simulink model "QD2_DroneStack_PID_2021a"  (R2022a)
settings: Solver=ode1  StartTime=0.0  StopTime=inf  FixedStep=1/1000  RelTol=1e-3  EnableMultiTasking=on
InitFcn:
  | Motor_Mapping_7_Inch
model workspace (MAT data in the model file):
  target_system = 1
values from neighbouring files (symbols this model uses):
  KT = [0.03616,0.117,-0.01215]    [Motor_Mapping_7_Inch.m]
  Motor_Matrix = [ 0.25   -1/(2*L_Roll)    1/(2*L_Pitch)    K_Tau/4;                  0.25   -1/(2*L_Roll)   -1/(2*L_Pitch)   -K_Tau/4;                  0.25    1/(2*L_Roll)    1/(2*L_Pitch)   -K_Tau/4;                  0.25    1/(2*L_Roll)   -1/(2*L_Pitch)    K_Tau/4]    [Motor_Mapping_7_Inch.m]
undefined symbols (not defined in the file or in its folder): _Commander, _QDrone2, _Stabilizer, datetime, HIL, lf, log_, m, n, qc_get_step_size, s, saved_data
libraries: quarc_library x94, simulink x27, simulink_extras x9
(part 4 of 4)

== matlab function QD2_DroneStack_PID_2021a/COMMANDER (ANGLE MODE)/STATE MACHINE LOGIC ==
  data: E_Abort output; isArm output; pt_ARM_to_TAKEOFF_THROTTLE output; pt_TAKE_OFF_HEIGHT_TO_AUTOLAND output; pt_FLIGHT_TO_AUTOLAND output; current_state input; initializing input; Tracking_Issue input; Communication_Issue input; low_battery input; trigger_1 input; trigger_2 input; E_abort input; joystick_issue input; net_throttle_at_trim input; net_throttle_close_to_zero input; ctrl_throttle_close_to_zero input; take_off_successful input; flying_too_low input; flying_too_high input; close_to_ground input; pt_TAKEOFF_THROTTLE_TO_TAKEOFF_HEIGHT output; pt_TAKE_OFF_HEIGHT_TO_FLIGHT output; pt_AUTOLAND_TO_DISABLE output; pt_EMERGENCY_STOP_TO_DISABLE output; pt_EMERGENCY_ABORT_TO_DISABLE output; Error output; stop_model output; sensor_failed input
function [E_Abort, isArm, pt_ARM_to_TAKEOFF_THROTTLE, pt_TAKE_OFF_HEIGHT_TO_AUTOLAND, pt_FLIGHT_TO_AUTOLAND, pt_TAKEOFF_THROTTLE_TO_TAKEOFF_HEIGHT, pt_TAKE_OFF_HEIGHT_TO_FLIGHT, pt_AUTOLAND_TO_DISABLE, pt_EMERGENCY_STOP_TO_DISABLE, pt_EMERGENCY_ABORT_TO_DISABLE, Error, stop_model]...
    = SM_logic(current_state, initializing, Tracking_Issue, Communication_Issue, low_battery, trigger_1, trigger_2, E_abort, joystick_issue,...
    net_throttle_at_trim, net_throttle_close_to_zero, ctrl_throttle_close_to_zero, take_off_successful, flying_too_low, flying_too_high, close_to_ground, sensor_failed)

% Programmatic Logic Block
%
% Logic for the FSM is generated here based on a variety of signals.
% Mostly, logic to programmatically trigger the transition to either a 
% natural next state, or an Error state, is generated here.
%
% Last modified: March, 2020
%
% INPUTS:
% -------
% current_state = previous state of the FSM-------------------------------------------------- (#)         [1]
% initializing = signal representing that the system is initializing (first 5s + buffer)- - - (bool)      [1]
% comm = communication signal representing MAVLINK connection-------------------------------- (bool)      [1]
% peripheral = signal representing joystick and optitrack connection- - - - - - - - - - - - - (bool)      [2]
% low_battery = signal representing low battery---------------------------------------------- (bool)      [1]
% trigger_1 = trigger representing ARM/DISARM - - - - - - - - - - - - - - - - - - - - - - - - (bool)      [1]
% trigger_2 = trigger representing TAKEOFF/AUTOLAND------------------------------------------ (bool)      [1]
% motors_not_spinning = signal representing the motors not spinning - - - - - - - - - - - - - (bool)      [1]
% net_throttle_at_trim = trim throttle for the application drone ---------------------------- (bool)      [1]
% net_throttle_close_to_zero = net throttle is close to zero in emergency stop mode - - - - - (bool)      [1]
% ctrl_throttle_close_to_zero = ctrl throttle is close to zero in emergency stop mode - - - - (bool)      [1]
% take_off_successful = signal representing whether drone has taken-off successfully -------- (bool)      [1]
% flying_too_low = signal representing whether the drone's height is below threshold and cmd- (bool)      [1]
% flying_too_high = signal representing whether the drone's height is above threshold-------- (bool)      [1]
% close_to_ground = signal representing whether the drone is close to the ground to autoland- (bool)      [1]
% 
% OUTPUTS:
% --------
% Error = Whether an Error is issued or not                                                             (bool)    [1]
% E_Abort = fed through for ease of understanding flow (see STATE MACHINE TRANSITION BLOCK)             (bool)    [1]
% isArm = programmatic transition state                                                                 (bool)    [1]
% takeoff = fed through for ease of understanding flow (see STATE MACHINE TRANSITION BLOCK)             (bool)    [1]
% pt_ARM_to_TAKEOFF_THROTTLE = programmatic transition state BEGIN_STATE_TO_FINAL_STATE                 (bool)    [1]
% pt_TAKEOFF_THROTTLE_TO_TAKEOFF_HEIGHT = programmatic transition state BEGIN_STATE_TO_FINAL_STATE      (bool)    [1]
% pt_TAKE_OFF_HEIGHT_TO_AUTOLAND = programmatic transition state BEGIN_STATE_TO_FINAL_STATE             (bool)    [1]
% pt_TAKEOFF_THROTTLE_TO_TAKEOFF_HEIGHT = programmatic transition state BEGIN_STATE_TO_FINAL_STATE      (bool)    [1]
% pt_TAKE_OFF_HEIGHT_TO_FLIGHT = programmatic transition state BEGIN_STATE_TO_FINAL_STATE               (bool)    [1]
% pt_AUTOLAND_TO_DISABLE = programmatic transition state BEGIN_STATE_TO_FINAL_STATE                     (bool)    [1]
% pt_EMERGENCY_STOP_TO_DISABLE = programmatic transition state BEGIN_STATE_TO_FINAL_STATE               (bool)    [1]
% pt_EMERGENCY_ABORT_TO_DISABLE = programmatic transition state BEGIN_STATE_TO_FINAL_STATE              (bool)    [1]
% stop_model = STOP THE MODEL AFTER                                                                     (bool)    [1]

Error = 0;
E_Abort = E_abort;
isArm = false;
pt_ARM_to_TAKEOFF_THROTTLE = false;
pt_TAKEOFF_THROTTLE_TO_TAKEOFF_HEIGHT = false;
pt_TAKE_OFF_HEIGHT_TO_AUTOLAND = false;
pt_TAKE_OFF_HEIGHT_TO_FLIGHT = false;
pt_FLIGHT_TO_AUTOLAND = false;
pt_AUTOLAND_TO_DISABLE = false;
pt_EMERGENCY_STOP_TO_DISABLE = false;
pt_EMERGENCY_ABORT_TO_DISABLE = false;
stop_model = 0;

switch current_state
    %---------------------------------------------------------------------%
    case 1 % IDLE STATE
        if (Communication_Issue)||...          % Communication issue
           (joystick_issue)||...               % joystick issue
           (Tracking_Issue)||...               % optitrack issue
           (low_battery)||...                  % low batter  
           (sensor_failed)||...                % if sensor (IMU) failure is detected on drone stabilizer    
           ((trigger_1)&&(initializing))||...  % armed while initializing
           (trigger_2)||...                    % tried to takeoff while initializing
           (~ctrl_throttle_close_to_zero)      % if throttle isn't at zero, don't arm
           %----------------------------------------%
            Error = 1;
        elseif trigger_1 % user arms
            isArm = true;
        end
    %---------------------------------------------------------------------%    
    case 2 % ARMED STATE
        isArm = trigger_1;
        if (Communication_Issue)||...          % Communication issue
           (joystick_issue)||...               % joystick issue
           (Tracking_Issue)||...               % optitrack issue
           (low_battery)||...                  % low battery
           (sensor_failed)||...                % if sensor (IMU) failure is detected on drone stabilizer
           (~ctrl_throttle_close_to_zero)      % if throttle isn't at zero, don't arm
           %----------------------------------------%
            Error = 1;
        elseif trigger_1 && trigger_2
            pt_ARM_to_TAKEOFF_THROTTLE = true;
        end        
    %---------------------------------------------------------------------%
    case 3 % TAKEOFF_THROTTLE STATE
        if (Communication_Issue)||...     % Communication issue
           (joystick_issue)||...          % joystick issue
           (Tracking_Issue)||...          % optitrack issue           
           (low_battery)||...             % low battery
           (sensor_failed)||...           % if sensor (IMU) failure is detected on drone stabilizer
           (~trigger_1)||...              % user disarms
           (~trigger_2)||...              % user commands auto-land before drone starts taking off
           (~ctrl_throttle_close_to_zero) % if throttle isn't at zero, don't arm
           %----------------------------------------%
            Error = 1;
        elseif net_throttle_at_trim
            pt_TAKEOFF_THROTTLE_TO_TAKEOFF_HEIGHT = true;
        end
    %---------------------------------------------------------------------%
    case 4 % TAKEOFF_HEIGHT STATE
        if (Communication_Issue)||... % Communication issue
           (joystick_issue)||...      % joystick issue
           (Tracking_Issue)||...      % optitrack issue
           (sensor_failed)||...       % if sensor (IMU) failure is detected on drone stabilizer    
           (flying_too_low)||...      % current height is below safety threshold 
           (flying_too_high)||...     % flying above safety margin (w.r.t optitrack)
           (~trigger_1)               % user disarms
            %----------------------------------------%
            Error = 1;
        elseif (~trigger_2)||low_battery 
            pt_TAKE_OFF_HEIGHT_TO_AUTOLAND = true;
        elseif take_off_successful
            pt_TAKE_OFF_HEIGHT_TO_FLIGHT = true;
        end
    %---------------------------------------------------------------------%
    case 5 % FLIGHT STATE
        if (Communication_Issue)||...   % Communication issue
           (joystick_issue)||...        % joystick issue
           (Tracking_Issue)||...        % optitrack issue
           (sensor_failed)||...         % if sensor (IMU) failure is detected on drone stabilizer
           (flying_too_low)||...        % current height is below safety threshold  
           (flying_too_high)||...       % flying above safety margin (w.r.t optitrack)
           (~trigger_1)                 % user disarms
           %----------------------------------------%
            Error = 1;
        elseif (~trigger_2)||low_battery
            pt_FLIGHT_TO_AUTOLAND = true;
        end
    %---------------------------------------------------------------------%
    case 6 % AUTOLAND STATE
        if (Communication_Issue)||...  % Communication issue
           (joystick_issue)||...       % joystick issue
           (Tracking_Issue)||...       % optitrack issue
           (sensor_failed)||...        % if sensor (IMU) failure is detected on drone stabilizer
           (flying_too_high)||...      % flying above safety margin (w.r.t optitrack)    
           (~trigger_1)                % user disarms
           %----------------------------------------%
            Error = 1;
        elseif close_to_ground 
            pt_AUTOLAND_TO_DISABLE = true;
        end
    %---------------------------------------------------------------------%
    case 7 % EMERGENCY LAND STATE
        if net_throttle_close_to_zero 
            pt_EMERGENCY_STOP_TO_DISABLE = true;
        end
    %---------------------------------------------------------------------%
    case 8 % EMERGENCY ABORT STATE
        pt_EMERGENCY_ABORT_TO_DISABLE = true;
    %---------------------------------------------------------------------%
    case 9
        % Stop the model.
        stop_model = 1;
end

== matlab function QD2_DroneStack_PID_2021a/COMMANDER (ANGLE MODE)/STATE MACHINE TRANSITION ==
  data: current_state input; E_Abort input; isArm input; pt_ARM_to_TAKEOFF_THROTTLE input; pt_TAKE_OFF_HEIGHT_TO_AUTOLAND input; pt_FLIGHT_TO_AUTOLAND input; Next_state output; pt_TAKEOFF_THROTTLE_TO_TAKEOFF_HEIGHT input; pt_TAKE_OFF_HEIGHT_TO_FLIGHT input; pt_AUTOLAND_TO_DISABLE input; pt_EMERGENCY_STOP_TO_DISABLE input; pt_EMERGENCY_ABORT_TO_DISABLE input; Error input
function Next_state = SM_transition(current_state, E_Abort, isArm, pt_ARM_to_TAKEOFF_THROTTLE, pt_TAKE_OFF_HEIGHT_TO_AUTOLAND, pt_FLIGHT_TO_AUTOLAND, pt_TAKEOFF_THROTTLE_TO_TAKEOFF_HEIGHT, pt_TAKE_OFF_HEIGHT_TO_FLIGHT, pt_AUTOLAND_TO_DISABLE, pt_EMERGENCY_STOP_TO_DISABLE, pt_EMERGENCY_ABORT_TO_DISABLE, Error)

% Programmatic Transition Block
%
% FINITE STATE MACHINE (FSM) with 9 states as described below, transitioning based on the 
% values of the isArm, transition signals, Error, and E_Abort
%
% Last modified: March, 2020
%
% INPUTS:
% ------
% current_state = Current state of the FSM        (#)     [1]
% E_Abort                                         (bool)  [1]
% isArm                                           (bool)  [1]
% pt_ARM_TO_TAKEOFF_THROTTLE                      (bool)  [1]
% pt_TAKE_OFF_HEIGHT_TO_AUTOLAND                  (bool)  [1]
% pt_FLIGHT_TO_AUTOLAND                           (bool)  [1]
% pt_TAKEOFF_THROTTLE_TO_TAKEOFF_HEIGHT           (bool)  [1]
% pt_TAKE_OFF_HEIGHT_TO_FLIGHT                    (bool)  [1]
% pt_AUTOLAND_TO_DISABLE                          (bool)  [1]
% pt_EMERGENCY_STOP_TO_DISABLE                    (bool)  [1]
% pt_EMERGENCY_ABORT_TO_DISABLE                   (bool)  [1]
% Error                                           (bool)  [1]
%
% OUTPUT:
% -------
% Next_state = Next state of the FSM              (#)     [1]

Next_state = double(0);
switch current_state
%-------------------------------------------------------------------------%
    case 1 % IDLE STATE
        if E_Abort
            Next_state = 8; % GOTO EMERGENCY ABORT STATE
        elseif Error
            Next_state = 7; % GOTO EMERGENCY STOP STATE
        elseif isArm
            Next_state = 2; % GOTO ARMED STATE
        else
            Next_state = 1; % STAY IN IDLE STATE
        end
%-------------------------------------------------------------------------%
    case 2 % ARMED STATE
        if E_Abort
            Next_state = 8; % GOTO EMERGENCY ABORT STATE
        elseif Error
            Next_state = 7; % GOTO EMERGENCY STOP STATE
        elseif ~isArm
            Next_state = 1; % GOTO IDLE STATE
        elseif pt_ARM_to_TAKEOFF_THROTTLE
            Next_state = 3; % GOTO TAKEOFF_THROTTLE STATE 
        else
            Next_state = 2; % STAY IN ARMED STATE
        end
%-------------------------------------------------------------------------%
    case 3 % TAKEOFF_THROTTLE STATE
        if E_Abort
            Next_state = 8; % GOTO EMERGENCY ABORT STATE
        elseif Error
            Next_state = 7; % GOTO EMERGENCY STOP STATE
        elseif pt_TAKEOFF_THROTTLE_TO_TAKEOFF_HEIGHT
            Next_state = 4; % GOTO TAKEOFF_HEIGHT STATE
        else
            Next_state = 3; % STAY IN TAKEOFF_THROTTLE STATE
        end
%-------------------------------------------------------------------------%
    case 4 % TAKEOFF_HEIGHT STATE
        if E_Abort
            Next_state = 8; % GOTO EMERGENCY ABORT STATE
        elseif Error
            Next_state = 7; % GOTO EMERGENCY STOP STATE
        elseif pt_TAKE_OFF_HEIGHT_TO_AUTOLAND
            Next_state = 6;
        elseif pt_TAKE_OFF_HEIGHT_TO_FLIGHT
            Next_state = 5; % GOTO FLIGHT STATE
        else
            Next_state = 4; % STAY IN TAKEOFF_HEIGHT STATE
        end
%-------------------------------------------------------------------------%
    case 5 % FLIGHT STATE
        if E_Abort
            Next_state = 8; % GOTO EMERGENCY ABORT STATE
        elseif Error
            Next_state = 7; % GOTO EMERGENCY STOP STATE
        elseif pt_FLIGHT_TO_AUTOLAND
            Next_state = 6; % GOTO AUTO_LAND STATE
        else
            Next_state = 5; % STAY IN FLIGHT STATE
        end
%-------------------------------------------------------------------------%       
    case 6 % AUTO_LAND STATE
        if E_Abort
            Next_state = 8; % GOTO EMERGENCY ABORT STATE
        elseif Error
            Next_state = 7; % GOTO EMERGENCY STOP STATE
        elseif pt_AUTOLAND_TO_DISABLE
            Next_state = 9; % GOTO DISABLE STATE
        else
            Next_state = 6; % STAY IN AUTO_LAND STATE
        end
%-------------------------------------------------------------------------%
    case 7 % EMERGENCY STOP STATE
        if E_Abort
            Next_state = 8; % GOTO EMERGENCY ABORT STATE
        elseif pt_EMERGENCY_STOP_TO_DISABLE
            Next_state = 9; % GOTO DISABLE STATE
        else
            Next_state = 7; % STAY IN EMERGENCY STOP STATE
        end
%-------------------------------------------------------------------------%
    case 8 % EMERGENCY ABORT
        if pt_EMERGENCY_ABORT_TO_DISABLE
            Next_state = 9; % GOTO DISABLE STATE
        else 
            Next_state = 8; % STAY IN EMERGENCY ABORT STATE
        end
%-------------------------------------------------------------------------%    
    case 9 % DISABLE
        Next_state = 9; % Always stay in DISABLE state if you are here    
end

== matlab function QD2_DroneStack_PID_2021a/Communication/Detect Communication Loss/MATLAB Function ==
  settings: updateMethod=DISCRETE
  data: time input; stream_connection_loss output; state input; error input; ms_time input; data_loss output
function [stream_connection_loss , data_loss] = fcn(time, state, error, ms_time)

persistent ms_time_prev
    if isempty(ms_time_prev)
        ms_time_prev = 0;
    end

stream_connection_loss = 0;
data_loss = 0;
if time > 3
    if ((state ~= 2)&&(error < 0))
        % stream connection is not established correctly
        stream_connection_loss = 1;
    end

    if (ms_time == ms_time_prev)&&(ms_time > 0)
        % data is stale
        data_loss = 1;
    end
end

ms_time_prev = ms_time;

== matlab function QD2_DroneStack_PID_2021a/QDrone2 DAQ/Force to percentage Mapping ==
  data: V_Bat_Act input; Motor_Forces input; Duty_Cycle output; KT input
function Duty_Cycle = fcn(V_Bat_Act,Motor_Forces,KT)

B = KT(2)^2-4*KT(1)*(KT(3)-Motor_Forces)

invalid_signal = B < 0
B(invalid_signal) = 0

% Ranges from 1000-2000
Volt_CMD_Theo = -0.5*KT(2)/KT(1)+ sqrt(B)/(2*KT(1));

Duty_Cycle = Volt_CMD_Theo/V_Bat_Act;

== matlab function QD2_DroneStack_PID_2021a/QDrone2 DAQ/Attitude Estimate from IMU Data/For Each Subsystem - Attitutde Estimates/roll and pitch approximation from accelerometer ==
  data: roll_acc output; pitch_acc output; acc_body input
function [roll_acc, pitch_acc]   = fcn(acc_body)
%#eml
n = norm(acc_body,2);
if n>eps
    acc_body = acc_body/n; 
else
    acc_body = [0 0 1]';
end

roll_acc = atan2(acc_body(2),acc_body(3));
pitch_acc = atan2( -acc_body(1), acc_body(2)*sin(roll_acc)+acc_body(3)*cos(roll_acc));

== matlab function QD2_DroneStack_PID_2021a/QDrone2 DAQ/Subsystem/MATLAB Function LED Color Assignment ==
  data: E_Stop input; Arm input; value output; low_battery input
function value = fcn(E_Stop, Arm, low_battery)

if low_battery == 1|| E_Stop ==1
    value = 1;
elseif Arm == 1 & E_Stop ==0
    value = 2;
elseif Arm == 0 && E_Stop == 0 
    value = 3;
else 
    value = 3;
end

== matlab function QD2_DroneStack_PID_2021a/COMMANDER (ANGLE MODE)/THROTTLE SWITCHBOX /Throttle Switchbox ==
  data: FSM_state input; sigmoid output
function sigmoid  = application_drone_throttle_switchbox(FSM_state)

% Application Drone: Throttle Switchbox
%
% Logic for switching between throttle commands from the controller 
%
% v2.0 - 5th october, 2018
%
% INPUTS:
% -------
% FSM_state = current state of the FSM------------------------------------------------------- (#)         [1]
% 
% OUTPUTS:
% --------
% sigmoid = an integer whose state determines how the heights are transformed---------------- (#)         [1]
% sigmoid = 1 - Command 0 throttle
% sigmoid = 2 - Sigmoid throttle up from 0 to the trim value
% sigmoid = 3 - Pass controller throttle straight through + trim value.
% sigmoid = 4 - Ignore controller throttle. Sigmoid it down to 0.
% sigmoid = 5 - Pass controller throttle straight through + trim value.


sigmoid = 0;
switch FSM_state
    case 1 % IDLE STATE
        sigmoid = 1;
    case 2 % ARM STATE
        sigmoid = 1;
    case 3 % TAKEOFF THROTTLE STATE
        sigmoid = 2;
    case 4 % TAKEOFF HEIGHT STATE
        sigmoid = 3;
    case 5 % FLIGHT STATE
        sigmoid = 3;
    case 6 % AUTOLAND STATE
        sigmoid = 5;
    case 7 % EMERGENCY STOP STATE
        sigmoid = 4;
    case 8 % EMERGENCY ABORT STATE
        sigmoid = 1;
    case 9 % DISABLE STATE
        sigmoid = 1;
end

== matlab function QD2_DroneStack_PID_2021a/QDrone2 DAQ/MotorCMD_FSM ==
  data: Arm_Signal input; E_Stop input; ESC_cmd output; Motor_State output; Model_Time input; Motor_State input
function [ESC_cmd,Motor_State]= fcn(Arm_Signal,E_Stop,Model_Time, Motor_State)

persistent state ESC_CMD 

%  Initialize motor state at the start of the model
if isempty(state)
    state = 2;
    ESC_CMD = zeros(1,4);
end 

% ESC Numbers w.r.t motor positions on QDrone: 
%         FRONT
%       4(3)       2(1)
% 
%       3(2)       1(0)
%          BACK  


% ============ Motor programing state machine ============ 

% State machine transitions: 

% Motor configuration state: 
if E_Stop == 0 && state ~= 9
    % Start with the motors in an idle state    
    if state == 2 && Model_Time > 0 && Model_Time <= 1  
        if Arm_Signal == 1
            % Error state, you started the model while the QDrone was armed
            state = 9;
        end 
           
    elseif state ==2  && Model_Time > 1 && Model_Time <= 2
        % Enter motor Low Frequency state:
        state = 1;
        
    elseif state ==1  && Model_Time > 2 && Model_Time <= 2.5
        % Set motor orientation
        state = 0;
        
    elseif state == 0 && Model_Time > 2.5    
        % Enter motor idle state: 
        state = 2; 

    elseif Motor_State ==2 && Arm_Signal == 1 
        % Enter arm state 
        state = 3;

    elseif Motor_State ==3 && Arm_Signal ==0 
        % Return to idle state 
        state = 2; 
    end 
    
elseif E_Stop ==1 
    % You've entered emergency state, disarm QDrone2!
    state = 9; 
end 


% State Machine commands: 
switch state 
    
    % ESC orientation set:
    case 0
        % for all drones
        ESC_CMD = [20,21,21,20];
        %for 1st R&D Drone 
        % ESC_CMD = [0,0,0,0];
    
    % Motor Low Frequency Beep:
    case 1
        ESC_CMD = [1,1,1,1];
    
    % Enter motor stop state: 
    case 2
        ESC_CMD = [0,0,0,0];
    
    % Motors in Arm State:
    case 3
        ESC_CMD = [48,48,48,48];
        
    % Same as state 2 but used as an Error State to stop motor cmd:
    case 9
        ESC_CMD = [0,0,0,0];
        
end 
    


Motor_State = state;
ESC_cmd = ESC_CMD;

Motor_State, ESC_cmd;

== matlab function QD2_DroneStack_PID_2021a/HORIZON FRAME CONVERSION AND ESTIMATION/Pose Switchbox/MATLAB Function ==
  data: sigmoid_type input; enable output; x_des input; slow_lim input; fast_lim input; x_cur input; x_vel input; x_ref output; max_x_vel output; max_x_accel output; x_meas input
function [enable, x_ref, max_x_vel, max_x_accel] = fcn(sigmoid_type, x_des, slow_lim, fast_lim, x_cur, x_vel, x_meas)

% Note: Some of the cases below are identical. However, they are separated out 
% based on the states of the state machine for ease of modification in the future. 
% For example, states 4 and 5 are identical. However, if the user wants different 
% signmoid behaviour when taking off than when landing, these cases may not be the same. 

enable = 0;
x_ref = 0;
max_x_vel = 0;
max_x_accel = 0;

switch sigmoid_type
    case 1 % This is for the IDLE, ARM, E_ABORT, E_STOP and DISABLE states of the FSM
        enable = 1;
        x_ref = x_meas;
        max_x_vel = slow_lim(1);
        max_x_accel = slow_lim(2);

    case 2 % This is for the TAKEOFF THROTTLE state of the FSM
        enable = 1;
        x_ref = x_meas;
        max_x_vel = slow_lim(1);
        max_x_accel = slow_lim(2);

    case 3 % This is for the FLIGHT state of the FSM
        enable = 1;
        x_ref = x_des;
        max_x_vel = fast_lim(1);
        max_x_accel = fast_lim(2);

    case 4 % This is for the TAKEOFF HEIGHT state of the FSM
        enable = 1;
        x_ref = x_des;
        if (abs(x_cur - x_des) <= 0.02)
            max_x_vel = fast_lim(1);
            max_x_accel = fast_lim(2);
        else    
            max_x_vel = slow_lim(1);
            max_x_accel = slow_lim(2);
        end
    case 5 % This is for the AUTOLAND state of the FSM
        enable = 1;
        x_ref = x_des;
        if (abs(x_cur - x_des) <= 0.02)
            max_x_vel = fast_lim(1);
            max_x_accel = fast_lim(2);        
        else
            max_x_vel = slow_lim(1);
            max_x_accel = slow_lim(2);
        end
        
end

== matlab function QD2_DroneStack_PID_2021a/HORIZON FRAME CONVERSION AND ESTIMATION/Pose Switchbox/MATLAB Function1 ==
  data: sigmoid_type input; enable output; y_des input; slow_lim input; fast_lim input; y_cur input; y_vel input; y_ref output; max_y_vel output; max_y_accel output; y_meas input
function [enable, y_ref, max_y_vel, max_y_accel] = fcn(sigmoid_type, y_des, slow_lim, fast_lim, y_cur, y_vel, y_meas)

% Note: Some of the cases below are identical. However, they are separated out 
% based on the states of the state machine for ease of modification in the future. 
% For example, states 4 and 5 are identical. However, if the user wants different 
% signmoid behaviour when taking off than when landing, these cases may not be the same. 

enable = 0;
y_ref = 0;
max_y_vel = 0;
max_y_accel = 0;

switch sigmoid_type
    case 1 % This is for the IDLE, ARM, E_ABORT, E_STOP and DISABLE states of the FSM
        enable = 1;
        y_ref = y_meas;
        max_y_vel = slow_lim(1);
        max_y_accel = slow_lim(2);

    case 2 % This is for the TAKEOFF THROTTLE state of the FSM
        enable = 1;
        y_ref = y_meas;
        max_y_vel = slow_lim(1);
        max_y_accel = slow_lim(2);

    case 3 % This is for the FLIGHT state of the FSM
        enable = 1;
        y_ref = y_des;
        max_y_vel = fast_lim(1);
        max_y_accel = fast_lim(2);

    case 4 % This is for the TAKEOFF HEIGHT state of the FSM
        enable = 1;
        y_ref = y_des;
        if (abs(y_cur - y_des) <= 0.02)
            max_y_vel = fast_lim(1);
            max_y_accel = fast_lim(2);
        else    
            max_y_vel = slow_lim(1);
            max_y_accel = slow_lim(2);
        end
    case 5 % This is for the AUTOLAND state of the FSM
        enable = 1;
        y_ref = y_des;
        if (abs(y_cur - y_des) <= 0.02)
            max_y_vel = fast_lim(1);
            max_y_accel = fast_lim(2);        
        else
            max_y_vel = slow_lim(1);
            max_y_accel = slow_lim(2);
        end
        
end
